simulink model "LunarMicrogrid_Full"  (R2026b)
settings: Solver=ode23t  StopTime=simulation.timeSim  MaxStep=1/(5*solarPlant.converterSwitchingFrequency)  AbsTol=1e-3
PreLoadFcn:
  | run('LunarMicrogridA_Data');
values from neighbouring files (symbols this model uses):
  Csc = Csc_cell/Ns_sc*Np_sc    (= 200)    [LunarDAB_Params.m]
  eta_sc = 0.95    [LunarDAB_Params.m]
  fsw = 100e3    (= 100000)    [LunarDAB_Params.m]
  k_restore = 1    [LunarDAB_Params.m]
  kiCurrent = 2    [LunarDAB_Params.m]
  kiVoltage = 8    [LunarDAB_Params.m]
  kpCurrent = 0.005    [LunarDAB_Params.m]
  kpVoltage = 0.4    [LunarDAB_Params.m]
  lTotal = lSeries + Llk    [LunarDAB_Params.m]
  P170_dt = 1e-4    (= 0.0001)    [P170_PV_Initialize.m]
  P170_Imp = im(ix)    [P170_PV_Initialize.m]
  P170_Vmp = vm(ix)    [P170_PV_Initialize.m]
  Rd_bat = dV_droop/Ibat_max    (= 0.232258064516)    [LunarDAB_Params.m]
  SC_enable = 1    [LunarDAB_Params.m]
  thetaIC = 0    [LunarDAB_Params.m]
  thetaMaxDab = pi/4    (= 0.785398163397)    [LunarDAB_Params.m]
  Tsw = 1/fsw    (= 1e-05)    [LunarDAB_Params.m]
  Vsc0 = sqrt((Vsc_max^2 + Vsc_min^2)/2)    [LunarDAB_Params.m]
  Vsc_max = 119    [LunarDAB_Params.m]
  Vsc_min = 66    [LunarDAB_Params.m]
undefined symbols (not defined in the file or in its folder): a_lpf_sys, battery, bms, connectedLoad, dcVoltage, DiscIntNeverNeededParam, eta_dab, Ibat_sign, mmc, Ndab, P170_T, pvDroop, sc, sensor, socLimit, solarPlant
libraries: sl_discontinuities x13, fl_lib x13, nesl_utility x13, simulink x7, batteryecm_lib x1, simulink_extras x1, ee_lib x1
(part 1 of 8)
settings Model: Creator=The MathWorks, Inc.  LastModifiedBy=Samiya
settings SolverCC: AutoScaleAbsTol=off
settings DataIOCC: DSMLogging=off  ReturnWorkspaceOutputs=off  SaveOutput=off  SaveTime=off  SignalLoggingName=SolarPVDCWithBattery_logDB
settings OptimizationCC: ReuseModelBlockBuffer=off
settings DebuggingCC: SymbolicDimsDataTypeCodeGenerationDiagnostic=none
settings SFSimCC: CustomCodeUndefinedFunction=UseInterfaceOnly
settings RTWCC: DLArmComputeVersion=19.05
settings SimscapeCC: SimscapeLogName=simlog_SolarPVDCWithBattery  SimscapeLogSimulationStatistics=on  SimscapeLogType=all  SimscapeUseEnergyAccounting=off

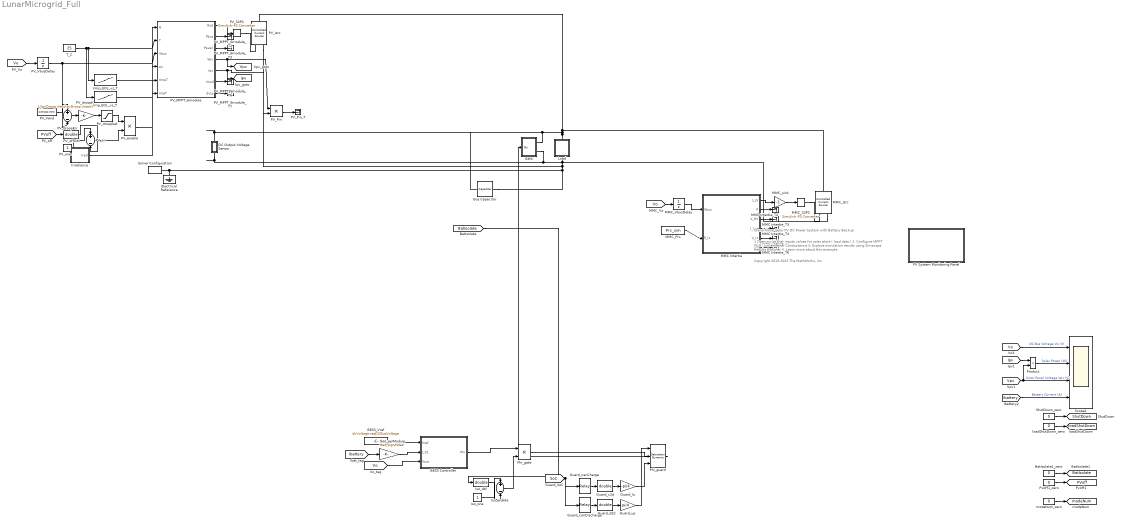
== system LunarMicrogrid_Full ==
  note: 1 Open script that inputs values for solar plant ( load data )
      | 2. Configure MPPT P&O , Incremental Conductance
      | 3. Explore simulation results using Simscape Results Explorer
      | 4. Learn more about this example
  note: Stand-Alone Solar PV DC Power System with Battery Backup
  note: Copyright 2019-2023 The MathWorks, Inc.
  BESS Controller : Subsystem
  BESS_Vref : Constant  Value=dcVoltage.reqDCBusVoltage
  BMS : Subsystem
  BatIsolate1_zero : Constant  Value=0  SampleTime=0
  Bus Capacitor : fl_lib/Electrical/Electrical Elements/Capacitor  c=boost.outputCapacitor F  r=1e-6 Ohm  g=0 1/Ohm  i_specify=off  i_priority=None  i=0 A  i_nominal_specify=off  i_nominal_value=1  i_nominal_unit=A  v_specify=off  v_priority=High  v=dcVoltage.reqDCBusVoltage V  v_nominal_specify=off  v_nominal_value=1  v_nominal_unit=V  vc_specify=on  vc_priority=High  vc=dcVoltage.reqDCBusVoltage V  vc_nominal_specify=off  vc_nominal_value=1  vc_nominal_unit=V
  DC Output Voltage Sensor : Subsystem
      mask Display: disp('v')
  Electrical Reference : fl_lib/Electrical/Electrical Elements/Electrical Reference
  Guard_c2d : DataTypeConversion  OutDataTypeStr=double  SaturateOnIntegerOverflow=off  RndMeth=Floor
  Guard_canCharge : Relay  OnSwitchValue=socLimit.max  OffSwitchValue=socLimit.rechargeBelow  OnOutputValue=0  OffOutputValue=1
  Guard_canDischarge : Relay  OnSwitchValue=socLimit.dischargeAbove  OffSwitchValue=socLimit.min
  Guard_d2d : DataTypeConversion  OutDataTypeStr=double  SaturateOnIntegerOverflow=off  RndMeth=Floor
  Guard_lo : Gain  Gain=-pi/4
  Guard_up : Gain  Gain=pi/4
  Ibat_perModule : Gain  Gain=Ibat_sign/Ndab
  Imp_EOL_vs_T : Lookup_n-D  NumberOfTableDimensions=1  BreakpointsForDimension1=P170_T  Table=P170_Imp  InternalRulePriority=Speed  RndMeth=Simplest
  Irradiance : Subsystem
  Iso_dbl : DataTypeConversion  OutDataTypeStr=double  SaturateOnIntegerOverflow=off  RndMeth=Floor
  Iso_enable : Sum  Inputs=+-
  Iso_one : Constant
  Load : Subsystem
  MMC Intertie : MATLAB Function  TreatAsAtomicUnit=on
  MMC Intertie_T{2..6} (5 alike) : Terminator
  MMC_Isrc : fl_lib/Electrical/Electrical Sources/Controlled Current Source
  MMC_Prx : FromWorkspace  VariableName=Prx_sim  Interpolate=off  OutputAfterFinalValue=Holding final value
  MMC_S2PS : nesl_utility/Simulink-PS Converter  PhysicalDomain=network_engine_domain  SubClassName=ps_input  LeftPortType=input  RightPortType=output  PseudoPeriodic=off  Frequencies=[]  NoiseDistribution=none  NoiseParameters=[]  Unit=1  AffineConversion=off  FilteringAndDerivatives=filter  SimscapeFilterOrder=1  InputFilterTimeConstant=1e-4  UdotUserProvided=0
  MMC_VbusDelay : UnitDelay  InitialCondition=dcVoltage.reqDCBusVoltage  SampleTime=mmc.dt
  MMC_sink : Gain  Gain=-1
  PV System Monitoring Panel : Subsystem
  PV_Isrc : fl_lib/Electrical/Electrical Sources/Controlled Current Source
  PV_MPPT_6module : MATLAB Function  TreatAsAtomicUnit=on
  PV_MPPT_6module_T{2..3,6..7} (4 alike) : Terminator
  PV_Pin : Product
  PV_Pin_T : Terminator
  PV_S2PS : nesl_utility/Simulink-PS Converter  PhysicalDomain=network_engine_domain  SubClassName=ps_input  LeftPortType=input  RightPortType=output  PseudoPeriodic=off  Frequencies=[]  NoiseDistribution=none  NoiseParameters=[]  Unit=1  AffineConversion=off  FilteringAndDerivatives=filter  SimscapeFilterOrder=1  InputFilterTimeConstant=1e-4  UdotUserProvided=0
  PV_VbusDelay : UnitDelay  InitialCondition=dcVoltage.reqDCBusVoltage  SampleTime=P170_dt
  PV_Vend : Constant  Value=pvDroop.Vend
  PV_droopErr : Sum  Inputs=+-
  PV_droopK : Gain  Gain=1/(pvDroop.Vend-pvDroop.Vstart)
  PV_droopSat : Saturate  UpperLimit=1  LowerLimit=0
  PV_enable : Product
  PV_offDbl : DataTypeConversion  OutDataTypeStr=double  SaturateOnIntegerOverflow=off  RndMeth=Floor
  PV_on : Sum  Inputs=+-
  PV_one : Constant
  Phi_gate : Product
  Phi_guard : sl_discontinuities/Saturation Dynamic  OutMin=[]  OutMax=[]  OutDataTypeStr=Inherit: Same as second input  OutDataType=fixdt(1, 16)  OutScaling=2^-10  DoSatur=off
      settings: LibrarySourceBlock=|
      | simulink/Discontinuities/Saturation
      | Dynamic
  Product : Product
  Pvoff1_zero : Constant  Value=0  SampleTime=0
  Scope1 : Scope  NumInputPorts=4
      settings: TimeSpan=simulation.timeSim  ActiveDisplayYMinimum=-72.27632  ActiveDisplayYMaximum=650.48692
  ShutDown_zero : Constant  Value=0  SampleTime=0
  Solver Configuration : nesl_utility/Solver Configuration  PhysicalDomain=network_engine_domain  SubClassName=solver  LeftPortType=input  RightPortType=generic  Tones=[]  Harmonics=[]  SimulateNoise=off  Profile=off  UseLocalSampling=off  EnableSwitchedLinearOptims=on  FrequencyDomain=off  UseCCode=off  RelTol=0.001  AbsTol=1e-06  MinStep=1e-09  ToWorkspace=off  RevertToSquareIcSolve=off  NumHomotopyIterations=100  PhasorMode=off  PhasorModeNumHarmonics=1  ConsistencySolver=NEWTON_FTOL  CanonicalOrdering=UNORDERED  OptimizeIntermediates=UNOPTIMIZED  MulticoreSolverChoice=BACKWARD_EULER  IndexReductionMethod=DerivativeReplacement  DoDC=off  ResidualTolerance=1e-9  ConsistencyTolSource=GLOBAL  ConsistencyAbsTol=0.001  ConsistencyRelTol=0.001  ConsistencyTolFactor=0.001  UseLocalSolver=off  LocalSolverChoice=NE_TRAPEZOIDAL_ADVANCER  ResolveIndetEquations=on  FunctionEvalNumThread=1  LocalSolverSampleTime=2e-6  DoFixedCost=off  MaxNonlinIter=10  MaxModeIter=2  ComputeImpulses=off  ImpulseIterations=2  LinearAlgebra=auto  LinearAlgebraNumThread=0  EquationFormulation=NE_TIME_EF  DelaysMemoryBudget=1024  AutomaticFiltering=on  FilteringTimeConstant=0.001  PartitionStorageMethod=AS_NEEDED  PartitionMemoryBudget=1024  PartitionMethod=FAST  MultibodyUseLocalSolver=off  MultibodyLocalSolverChoice=ODE1  MultibodyLocalSolverSampleTime=0.001
  T_C : Constant  Value=25
  Vmp_EOL_vs_T : Lookup_n-D  NumberOfTableDimensions=1  BreakpointsForDimension1=P170_T  Table=P170_Vmp  InternalRulePriority=Speed  RndMeth=Simplest
  loadShutDown_zero : Constant  Value=0  SampleTime=0
  modeNum_zero : Constant  Value=0  SampleTime=0
  tag scope: BatIsolate=global, Ipv=global, PVoff=global, ShutDown=global, Vpv=global, loadShutDown=global, modeNum=global
  wires:
  [Vpv] -> Scope1/3, Product/2  "Solar Panel Voltage Vpv (V)"
  Product/1 -> Scope1/2  "Solar Power (W)"
  [Ipv] -> Product/1
  [Vo] -> Scope1/1  "DC Bus Voltage Vo (V)"
  [Ibattery] -> Scope1/4  "Battery Current (A)"
  BESS_Vref/1 -> BESS Controller/1(Vref)
  [Ibattery] -> Ibat_perModule/1
  Ibat_perModule/1 -> BESS Controller/2(I_V1)
  [Vo] -> BESS Controller/3(Vout)
  [BatIsolate] -> Iso_dbl/1
  Iso_one/1 -> Iso_enable/1
  Iso_dbl/1 -> Iso_enable/2
  BESS Controller/1(Phi) -> Phi_gate/1
  Iso_enable/1 -> Phi_gate/2
  Irradiance/1(Irad) -> PV_MPPT_6module/1(G)
  T_C/1 -> PV_MPPT_6module/2(T), Vmp_EOL_vs_T/1, Imp_EOL_vs_T/1
  [Vo] -> PV_VbusDelay/1
  PV_VbusDelay/1 -> PV_MPPT_6module/3(Vbus), PV_droopErr/2
  PV_Vend/1 -> PV_droopErr/1
  PV_droopErr/1 -> PV_droopK/1
  PV_droopK/1 -> PV_droopSat/1
  [PVoff] -> PV_offDbl/1
  PV_one/1 -> PV_on/1
  PV_offDbl/1 -> PV_on/2
  PV_droopSat/1 -> PV_enable/1
  PV_on/1 -> PV_enable/2
  PV_enable/1 -> PV_MPPT_6module/4(en)
  Vmp_EOL_vs_T/1 -> PV_MPPT_6module/5(VmpT)
  Imp_EOL_vs_T/1 -> PV_MPPT_6module/6(ImpT)
  PV_MPPT_6module/1(Ibus) -> PV_S2PS/1
  PV_MPPT_6module/4(Vpv) -> [Vpv], PV_Pin/1
  PV_MPPT_6module/5(Ipv) -> [Ipv], PV_Pin/2
  [Vo] -> MMC_VbusDelay/1
  MMC_VbusDelay/1 -> MMC Intertie/1(Vbus)
  MMC Intertie/1(I_LV) -> MMC_sink/1
  MMC_sink/1 -> MMC_S2PS/1
  PV_MPPT_6module/2(Pbus) -> PV_MPPT_6module_T2/1
  PV_MPPT_6module/3(Pavail) -> PV_MPPT_6module_T3/1
  PV_MPPT_6module/6(Imod) -> PV_MPPT_6module_T6/1
  PV_MPPT_6module/7(duty) -> PV_MPPT_6module_T7/1
  MMC Intertie/2(P) -> MMC Intertie_T2/1
  MMC Intertie/3(V_HV) -> MMC Intertie_T3/1
  MMC Intertie/4(I_line) -> MMC Intertie_T4/1
  MMC Intertie/5(V_rx) -> MMC Intertie_T5/1
  MMC Intertie/6(phi) -> MMC Intertie_T6/1
  PV_Pin/1 -> PV_Pin_T/1
  MMC_Prx/1 -> MMC Intertie/2(P_rx)
  ShutDown_zero/1 -> [ShutDown]
  loadShutDown_zero/1 -> [loadShutDown]
  BatIsolate1_zero/1 -> [BatIsolate]
  Pvoff1_zero/1 -> [PVoff]
  modeNum_zero/1 -> [modeNum]
  [SoC] -> Guard_canCharge/1, Guard_canDischarge/1
  Guard_c2d/1 -> Guard_lo/1
  Guard_d2d/1 -> Guard_up/1
  Guard_up/1 -> Phi_guard/1
  Phi_gate/1 -> Phi_guard/2
  Guard_lo/1 -> Phi_guard/3
  Phi_guard/1 -> BMS/1(Phi)
  Guard_canCharge/1 -> Guard_c2d/1
  Guard_canDischarge/1 -> Guard_d2d/1
  connections:
  BMS/RConn1 -- DC Output Voltage Sensor/RConn1 -- MMC_Isrc/LConn1 -- PV_Isrc/LConn1 -- Bus Capacitor/LConn1 -- Load/LConn1
  BMS/RConn2 -- Load/RConn1 -- Solver Configuration/RConn1 -- Electrical Reference/LConn1 -- Bus Capacitor/RConn1 -- PV_Isrc/RConn2 -- MMC_Isrc/RConn2 -- DC Output Voltage Sensor/LConn1
  PV_S2PS/RConn1 -- PV_Isrc/RConn1
  MMC_S2PS/RConn1 -- MMC_Isrc/RConn1
